simulink model "C1_Full_Car_Model"  (R2023b)
settings: Solver=FixedStepAuto  StartTime=0.0  StopTime=t_end_sim  FixedStep=Ts_sim  RelTol=1e-3
values from neighbouring files (symbols this model uses):
  a_b_ref_sat = [ zeros(1,10) ... (first row only)    [A1_Init.m]    (also in C1_MonteCarloAnalysis.m)
  adaptive = 3    [A1_Init.m]    (also in C1_MonteCarloAnalysis.m = 1)
  data = A2_Full_car_model_parameters_4onBoard()    [A1_Init.m]    (also in C1_MonteCarloAnalysis.m)
  Ft_demand_F = [zeros(1,601) 200*ones(1,2400)]./data.R_F    [A1_Init.m]    (also in C1_MonteCarloAnalysis.m)
  Ft_demand_R = [zeros(1,(601-length(l_discr)))              200*ones(1,(2400+length(l_discr)))]./data.R_R    [A1_Init.m]    (also in C1_MonteCarloAnalysis.m)
  handmade_front = strcat(currentPath,'\Road_profiles\height_crg_files\','handmade_step_3cm_singlefunctions.crg')    [A1_Init.m]    (also in C1_MonteCarloAnalysis.m)
  handmade_mu_front = strcat(currentPath,'\Road_profiles\friction_crg_files\','handmade_fric_step_01_singlefunctions.crg')    [A1_Init.m]    (also in C1_MonteCarloAnalysis.m)
  handmade_mu_rear = handmade_mu_front    [A1_Init.m]    (also in C1_MonteCarloAnalysis.m)
  handmade_rear = handmade_front    [A1_Init.m]    (also in C1_MonteCarloAnalysis.m)
  k_mu = mu_prev_scal_fact(i)    [C1_MonteCarloAnalysis.m]
  k_r = road_height_prev_scal_fact(i)    [C1_MonteCarloAnalysis.m]
  LowLim_Q1 = -10    [A1_Init.m]    (also in C1_MonteCarloAnalysis.m)
  M = N    (= 10)    [A1_Init.m]    (also in C1_MonteCarloAnalysis.m)
  mu_distance = test_distance    [A1_Init.m]    (also in C1_MonteCarloAnalysis.m)
  mu_road = [ones(1,1001), 0.1*ones(1,2000)]    [A1_Init.m]    (also in C1_MonteCarloAnalysis.m)
  N = 10    [A1_Init.m]    (also in C1_MonteCarloAnalysis.m)
  N_iter = 3    [A1_Init.m]    (also in C1_MonteCarloAnalysis.m)
  omega_ini_F_L = x_u_dot_ini_F_L/data.R_F    [A1_Init.m]    (also in C1_MonteCarloAnalysis.m)
  omega_ini_F_R = x_u_dot_ini_R_R/data.R_F    [A1_Init.m]    (also in C1_MonteCarloAnalysis.m)
  omega_ini_R_L = x_u_dot_ini_R_L/data.R_R +2.483*1e-6    [A1_Init.m]    (also in C1_MonteCarloAnalysis.m)
  omega_ini_R_R = x_u_dot_ini_R_R/data.R_R+2.483*1e-6    [A1_Init.m]    (also in C1_MonteCarloAnalysis.m)
  passive = 2    [A1_Init.m]    (also in C1_MonteCarloAnalysis.m)
  Pitch = 0    [A1_Init.m]    (also in C1_MonteCarloAnalysis.m)
  Pitch_dot = 0    [A1_Init.m]    (also in C1_MonteCarloAnalysis.m)
  preview = 2    [A1_Init.m]    (also in C1_MonteCarloAnalysis.m)
  Q1 = 1e6    (= 1000000)    [A1_Init.m]    (also in C1_MonteCarloAnalysis.m)
  Q1_sat = 0    [A1_Init.m]    (also in C1_MonteCarloAnalysis.m)
  Q2 = 1e5    (= 100000)    [A1_Init.m]    (also in C1_MonteCarloAnalysis.m)
  QN1 = 0    [A1_Init.m]    (also in C1_MonteCarloAnalysis.m)
  QN2 = 0    [A1_Init.m]    (also in C1_MonteCarloAnalysis.m)
  R1 = 1e10    (= 10000000000)    [A1_Init.m]    (also in C1_MonteCarloAnalysis.m)
  r1_h0 = 0.99    [A1_Init.m]    (also in C1_MonteCarloAnalysis.m)
  r1_k = 1000    [A1_Init.m]    (also in C1_MonteCarloAnalysis.m)
  r1_max = 11    [A1_Init.m]    (also in C1_MonteCarloAnalysis.m)
  r1_min = -10    [A1_Init.m]    (also in C1_MonteCarloAnalysis.m)
  r2 = 2    [A1_Init.m]    (also in C1_MonteCarloAnalysis.m)
  R2 = 1e2    (= 100)    [A1_Init.m]    (also in C1_MonteCarloAnalysis.m)
  R2_rl = 2    [A1_Init.m]    (also in C1_MonteCarloAnalysis.m)
  road_profile = [zeros(1,801),ones(1,2200)*10*Step_selector]    [A1_Init.m]    (also in C1_MonteCarloAnalysis.m)
  T_distance = test_distance    [A1_Init.m]    (also in C1_MonteCarloAnalysis.m)
  T_hs_ini_F_L = 0    [A1_Init.m]    (also in C1_MonteCarloAnalysis.m)
  T_hs_ini_F_R = 0    [A1_Init.m]    (also in C1_MonteCarloAnalysis.m)
  T_hs_ini_R_L = 0    [A1_Init.m]    (also in C1_MonteCarloAnalysis.m)
  T_hs_ini_R_R = 0    [A1_Init.m]    (also in C1_MonteCarloAnalysis.m)
  test_distance = 0:0.01:30    [A1_Init.m]    (also in C1_MonteCarloAnalysis.m)
  theta_s_ini_F_L = 0    [A1_Init.m]    (also in C1_MonteCarloAnalysis.m)
  theta_s_ini_F_R = 0    [A1_Init.m]    (also in C1_MonteCarloAnalysis.m)
  theta_s_ini_R_L = 0    [A1_Init.m]    (also in C1_MonteCarloAnalysis.m)
  theta_s_ini_R_R = 0    [A1_Init.m]    (also in C1_MonteCarloAnalysis.m)
  theta_w_ini_F_L = -1.056*1e-2    (= -0.01056)    [A1_Init.m]    (also in C1_MonteCarloAnalysis.m)
  theta_w_ini_R_L = -1.056*1e-2    (= -0.01056)    [A1_Init.m]    (also in C1_MonteCarloAnalysis.m)
  Ts = 1e-3*[0 5 10 15 20 25 30 40 60 80 100]    [A1_Init.m]    (also in C1_MonteCarloAnalysis.m)
  w1_h0 = 0.0008    [A1_Init.m]    (also in C1_MonteCarloAnalysis.m)
  w1_k = 5000    [A1_Init.m]    (also in C1_MonteCarloAnalysis.m)
  w1_max = 9    [A1_Init.m]    (also in C1_MonteCarloAnalysis.m)
  w1_min = -10    [A1_Init.m]    (also in C1_MonteCarloAnalysis.m)
  w1_sat = 0.085    [A1_Init.m]    (also in C1_MonteCarloAnalysis.m)
  w2_h0 = 2    [A1_Init.m]    (also in C1_MonteCarloAnalysis.m)
  w2_inc = 0.05    [A1_Init.m]    (also in C1_MonteCarloAnalysis.m)
  w2_k = 10    [A1_Init.m]    (also in C1_MonteCarloAnalysis.m)
  w2_max = 5.3    [A1_Init.m]    (also in C1_MonteCarloAnalysis.m)
  w2_min = -10    [A1_Init.m]    (also in C1_MonteCarloAnalysis.m)
  Wmat_NMPC_init = [W(1,:) W(2,:) W(3,:) W(4,:)]    [A1_Init.m]    (also in C1_MonteCarloAnalysis.m)
  WNmat_NMPC_init = [WN(1,:) WN(2,:)]    [A1_Init.m]    (also in C1_MonteCarloAnalysis.m)
  X_0 = [z_b_dot_ini z_b_ini z_u_dot_ini_F_L z_u_ini_F_L x_b_dot_ini x_b_ini x_u_dot_ini_F_L x_u_ini_F_L          omega_ini_F_L theta_w_ini_F_L omega_ini_F_L theta_s_ini_F_L torque_ini_F_L]    [A1_Init.m]    (also in C1_MonteCarloAnalysis.m)
  x_b_dot_ini = speed_ini/3.6    (= 11.1111111111)    [A1_Init.m]    (also in C1_MonteCarloAnalysis.m)
  x_b_ini = data.b+pos_ini    [A1_Init.m]    (also in C1_MonteCarloAnalysis.m)
  x_err = road_prev_pos_err(i)    [C1_MonteCarloAnalysis.m]
  x_u_dot_ini_F_L = speed_ini/3.6 - 1.125*1e-4    (= 11.1109986111)    [A1_Init.m]    (also in C1_MonteCarloAnalysis.m)
  x_u_dot_ini_F_R = speed_ini/3.6 - 1.125*1e-4    (= 11.1109986111)    [A1_Init.m]    (also in C1_MonteCarloAnalysis.m)
  x_u_dot_ini_R_L = speed_ini/3.6 - 1.125*1e-4    (= 11.1109986111)    [A1_Init.m]    (also in C1_MonteCarloAnalysis.m)
  x_u_dot_ini_R_R = speed_ini/3.6 - 1.125*1e-4    (= 11.1109986111)    [A1_Init.m]    (also in C1_MonteCarloAnalysis.m)
  x_u_ini_F_L = data.a+data.b+pos_ini    [A1_Init.m]    (also in C1_MonteCarloAnalysis.m)
  x_u_ini_F_R = data.a+data.b+pos_ini    [A1_Init.m]    (also in C1_MonteCarloAnalysis.m)
  x_u_ini_R_L = pos_ini    (= 0)    [A1_Init.m]    (also in C1_MonteCarloAnalysis.m)
  x_u_ini_R_R = pos_ini    (= 0)    [A1_Init.m]    (also in C1_MonteCarloAnalysis.m)
  z_b_dot_ini = 0    [A1_Init.m]    (also in C1_MonteCarloAnalysis.m)
  z_b_ini = 0    [A1_Init.m]    (also in C1_MonteCarloAnalysis.m)
  z_u_dot_ini_F_L = 0    [A1_Init.m]    (also in C1_MonteCarloAnalysis.m)
  z_u_dot_ini_F_R = 0    [A1_Init.m]    (also in C1_MonteCarloAnalysis.m)
  z_u_dot_ini_R_L = 0    [A1_Init.m]    (also in C1_MonteCarloAnalysis.m)
  z_u_dot_ini_R_R = 0    [A1_Init.m]    (also in C1_MonteCarloAnalysis.m)
  z_u_ini_F_L = 0    [A1_Init.m]    (also in C1_MonteCarloAnalysis.m)
  z_u_ini_F_R = 0    [A1_Init.m]    (also in C1_MonteCarloAnalysis.m)
  z_u_ini_R_L = 0    [A1_Init.m]    (also in C1_MonteCarloAnalysis.m)
  z_u_ini_R_R = 0    [A1_Init.m]    (also in C1_MonteCarloAnalysis.m)
undefined symbols (not defined in the file or in its folder): Delay_step, road_with_noise
libraries: mfswift_library x8, rllib x4, simulink x4
(part 2 of 7)

== system C1_Full_Car_Model/PASSIVE ==
  BUS : Inport
  Bus Selector : BusSelector  OutputSignals=States.x_u_F_L,States.x_u_F_R,States.x_u_R_L,States.x_u_R_R
  F_t_req1 : Lookup_n-D  NumberOfTableDimensions=1  BreakpointsForDimension1=T_distance  Table=Ft_demand_F  InterpMethod=Linear Lagrange  InternalRulePriority=Speed  RndMeth=Simplest
  F_t_req2 : Lookup_n-D  NumberOfTableDimensions=1  BreakpointsForDimension1=T_distance  Table=Ft_demand_R  InterpMethod=Linear Lagrange  InternalRulePriority=Speed  RndMeth=Simplest
  F_t_req3 : Lookup_n-D  NumberOfTableDimensions=1  BreakpointsForDimension1=T_distance  Table=Ft_demand_R  InterpMethod=Linear Lagrange  InternalRulePriority=Speed  RndMeth=Simplest
  F_t_req4 : Lookup_n-D  NumberOfTableDimensions=1  BreakpointsForDimension1=T_distance  Table=Ft_demand_F  InterpMethod=Linear Lagrange  InternalRulePriority=Speed  RndMeth=Simplest
  Gain : Gain  Gain=data.R_F
  Gain1 : Gain  Gain=data.R_R
  Gain2 : Gain  Gain=data.R_R
  Gain3 : Gain  Gain=data.R_F
  Gain6 : Gain  Gain=1/data.R_F
  Gain7 : Gain  Gain=1/data.R_R
  To Workspace : ToWorkspace  VariableName=T_ref_front_sim  SaveFormat=Timeseries  SampleTime=-1
  To Workspace1 : ToWorkspace  VariableName=T_ref_rear_sim  SaveFormat=Timeseries  SampleTime=-1
  Tt_req_F_L1 : Outport  VectorParamsAs1DForOutWhenUnconnected=off
  Tt_req_F_R1 : Outport  Port=2  VectorParamsAs1DForOutWhenUnconnected=off
  Tt_req_R_L1 : Outport  Port=3  VectorParamsAs1DForOutWhenUnconnected=off
  Tt_req_R_R1 : Outport  Port=4  VectorParamsAs1DForOutWhenUnconnected=off
  tag scope: Ft_req_F=global, Ft_req_R=global
  wires:
  F_t_req1/1 -> Gain/1
  BUS/1 -> Bus Selector/1
  Bus Selector/3 -> F_t_req2/1  "<x_u_R_L>"
  F_t_req2/1 -> Gain1/1
  Bus Selector/1 -> F_t_req1/1  "<x_u_F_L>"
  F_t_req3/1 -> Gain2/1
  Bus Selector/4 -> F_t_req3/1  "<x_u_R_R>"
  Bus Selector/2 -> F_t_req4/1  "<x_u_F_R>"
  F_t_req4/1 -> Gain3/1
  Gain/1 -> Gain6/1, Tt_req_F_L1/1, To Workspace/1
  Gain3/1 -> Tt_req_F_R1/1
  Gain2/1 -> Gain7/1, Tt_req_R_R1/1, To Workspace1/1
  Gain7/1 -> [Ft_req_R]
  Gain1/1 -> Tt_req_R_L1/1
  Gain6/1 -> [Ft_req_F]

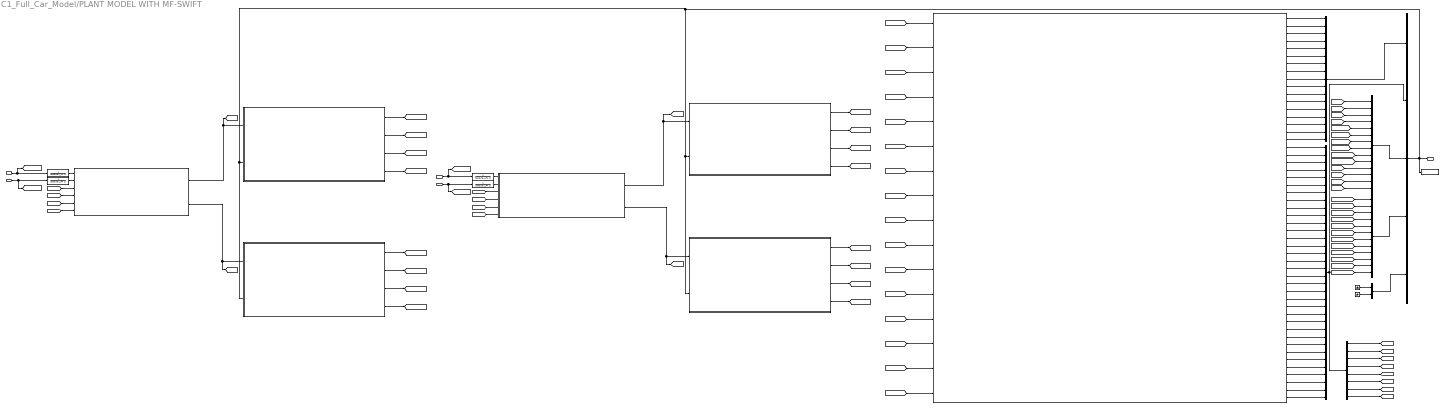
== system C1_Full_Car_Model/PLANT MODEL WITH MF-SWIFT ==
  Tm_F_L_req : Inport
  Tm_F_R_req : Inport  Port=2
  Tm_R_L_req : Inport  Port=3
  Tm_R_R_req : Inport  Port=4
  4 ON-BOARD POWERTRAIN - FRONT : Subsystem
  4 ON-BOARD POWERTRAIN - REAR : Subsystem
  Bus Creator : BusCreator  Inputs=12
  Bus Creator1 : BusCreator  Inputs=17
  Bus Creator2 : BusCreator  Inputs=34
  Bus Creator4 : BusCreator  Inputs=5
  Bus Creator5 : BusCreator  Inputs=14
  Bus Creator6 : BusCreator  Inputs=2
  Bus Selector1 : BusSelector  OutputSignals=omega_R_L,theta_R_L,omega_R_R,theta_R_R,omega_F_L,theta_F_L,omega_F_R,theta_F_R
  FRONT LEFT WHEEL : Subsystem
  FRONT RIGHT WHEEL : Subsystem
  Ground : Ground
  Ground1 : Ground
  MT dynamics1 : TransferFcn  Denominator=[data.tau_R4 1]
  MT dynamics2 : TransferFcn  Denominator=[data.tau_R4 1]
  MT dynamics3 : TransferFcn  Denominator=[data.tau_F4 1]
  MT dynamics4 : TransferFcn  Denominator=[data.tau_F4 1]
  REAR LEFT WHEEL : Subsystem
  REAR RIGHT WHEEL : Subsystem
  SUSPENSION MODEL : Subsystem
  To Workspace : ToWorkspace  VariableName=BUS  SaveFormat=Timeseries  SampleTime=-1
  BUS : Outport  VectorParamsAs1DForOutWhenUnconnected=off
  wires:
  [omega_F_L] -> 4 ON-BOARD POWERTRAIN - FRONT/4(omega_w_L)
  [omega_F_R] -> 4 ON-BOARD POWERTRAIN - FRONT/6(omega_w_R)
  [theta_F_R] -> 4 ON-BOARD POWERTRAIN - FRONT/5(theta_w_R)
  [theta_F_L] -> 4 ON-BOARD POWERTRAIN - FRONT/3(theta_w_L)
  [theta_R_R] -> 4 ON-BOARD POWERTRAIN - REAR/5(theta_w_R)
  [omega_R_R] -> 4 ON-BOARD POWERTRAIN - REAR/6(omega_w_R)
  [omega_R_L] -> 4 ON-BOARD POWERTRAIN - REAR/4(omega_w_L)
  [theta_R_L] -> 4 ON-BOARD POWERTRAIN - REAR/3(theta_w_L)
  [theta_s_ddot_F_R] -> Bus Creator/2  "theta_s_ddot_F_R"
  [theta_s_ddot_F_L] -> Bus Creator/1  "theta_s_ddot_F_L"
  [theta_s_ddot_R_R] -> Bus Creator/8  "theta_s_ddot_R_R"
  [theta_s_R_R] -> Bus Creator/12  "theta_s_R_R"
  [theta_s_R_L] -> Bus Creator/11  "theta_s_R_L"
  [theta_s_ddot_R_L] -> Bus Creator/7  "theta_s_ddot_R_L"
  [theta_s_F_R] -> Bus Creator/6  "theta_s_F_R"
  [theta_s_F_L] -> Bus Creator/5  "theta_s_F_L"
  [theta_s_dot_F_R] -> Bus Creator/4  "theta_s_dot_F_R"
  [theta_s_dot_F_L] -> Bus Creator/3  "theta_s_dot_F_L"
  Bus Creator/1 -> Bus Creator4/4  "Differentials"
  [T_hs_R_L] -> Bus Creator5/11  "T_hs_R_L"
  [T_hs_R_R] -> Bus Creator5/12  "T_hs_R_R"
  [T_hs_F_L] -> Bus Creator5/13  "T_hs_F_L"
  [T_hs_F_R] -> Bus Creator5/14  "T_hs_F_R"
  Bus Selector1/8 -> [theta_F_R]  "<theta_F_R>"
  Bus Selector1/7 -> [omega_F_R]  "<omega_F_R>"
  Bus Selector1/6 -> [theta_F_L]  "<theta_F_L>"
  Bus Selector1/5 -> [omega_F_L]  "<omega_F_L>"
  Bus Selector1/4 -> [theta_R_R]  "<theta_R_R>"
  Bus Selector1/1 -> [omega_R_L]  "<omega_R_L>"
  Bus Selector1/2 -> [theta_R_L]  "<theta_R_L>"
  Bus Selector1/3 -> [omega_R_R]  "<omega_R_R>"
  [Slip_F_R] -> SUSPENSION MODEL/16(Slip_F_R)
  [Rotational_F_R] -> SUSPENSION MODEL/15(Rotational_F_R)
  [Fz_F_R_tot] -> SUSPENSION MODEL/14(Fz_F_R_tot)
  [Fx_F_R] -> SUSPENSION MODEL/13(Fx_F_R)
  [Slip_F_L] -> SUSPENSION MODEL/12(Slip_F_L)
  [Rotational_F_L] -> SUSPENSION MODEL/11(Rotational_F_L)
  [Fz_F_L_tot] -> SUSPENSION MODEL/10(Fz_F_L_tot)
  [Fx_F_L] -> SUSPENSION MODEL/9(Fx_F_L)
  [Slip_R_R] -> SUSPENSION MODEL/8(Slip_R_R)
  [Rotational_R_R] -> SUSPENSION MODEL/7(Rotational_R_R)
  [Fz_R_R_tot] -> SUSPENSION MODEL/6(Fz_R_R_tot)
  [Fx_R_R] -> SUSPENSION MODEL/5(Fx_R_R)
  FRONT LEFT WHEEL/1(Fx_F_L) -> [Fx_F_L]
  FRONT LEFT WHEEL/2(Fz_F_L_tot) -> [Fz_F_L_tot]
  FRONT LEFT WHEEL/3(Rotational_F_L) -> [Rotational_F_L]
  FRONT LEFT WHEEL/4(Slip_F_L) -> [Slip_F_L]
  FRONT RIGHT WHEEL/4(Slip_F_R) -> [Slip_F_R]
  FRONT RIGHT WHEEL/3(Rotational_F_R) -> [Rotational_F_R]
  FRONT RIGHT WHEEL/2(Fz_F_R_tot) -> [Fz_F_R_tot]
  FRONT RIGHT WHEEL/1(Fx_F_R) -> [Fx_F_R]
  REAR RIGHT WHEEL/1(Fx_R_R) -> [Fx_R_R]
  REAR RIGHT WHEEL/2(Fz_R_R_tot) -> [Fz_R_R_tot]
  REAR RIGHT WHEEL/3(Rotational_R_R) -> [Rotational_R_R]
  REAR RIGHT WHEEL/4(Slip_R_R) -> [Slip_R_R]
  REAR LEFT WHEEL/4(Slip_R_L) -> [Slip_R_L]
  REAR LEFT WHEEL/3(Rotational_R_L) -> [Rotational_R_L]
  REAR LEFT WHEEL/2(Fz_R_L_tot) -> [Fz_R_L_tot]
  REAR LEFT WHEEL/1(Fx_R_L) -> [Fx_R_L]
  [Slip_R_L] -> SUSPENSION MODEL/4(Slip_R_L)
  [Rotational_R_L] -> SUSPENSION MODEL/3(Rotational_R_L)
  [Fz_R_L_tot] -> SUSPENSION MODEL/2(Fz_R_L_tot)
  [Fx_R_L] -> SUSPENSION MODEL/1(Fx_R_L)
  SUSPENSION MODEL/38(omega_R_L) -> Bus Creator2/21  "omega_R_L"
  SUSPENSION MODEL/37(x_u_F_R) -> Bus Creator2/20  "x_u_F_R"
  SUSPENSION MODEL/36(x_u_dot_F_R) -> Bus Creator2/19  "x_u_dot_F_R"
  SUSPENSION MODEL/35(x_u_F_L) -> Bus Creator2/18  "x_u_F_L"
  SUSPENSION MODEL/34(x_u_dot_F_L) -> Bus Creator2/17  "x_u_dot_F_L"
  SUSPENSION MODEL/51(slip_F_R) -> Bus Creator2/34  "slip_F_R"
  SUSPENSION MODEL/50(slip_F_L) -> Bus Creator2/33  "slip_F_L"
  SUSPENSION MODEL/49(slip_R_R) -> Bus Creator2/32  "slip_R_R"
  SUSPENSION MODEL/48(slip_R_L) -> Bus Creator2/31  "slip_R_L"
  SUSPENSION MODEL/47(pitch) -> Bus Creator2/30  "pitch"
  SUSPENSION MODEL/46(pitch_dot) -> Bus Creator2/29  "pitch_dot"
  SUSPENSION MODEL/45(theta_F_R) -> Bus Creator2/28  "theta_F_R"
  SUSPENSION MODEL/44(omega_F_R) -> Bus Creator2/27  "omega_F_R"
  SUSPENSION MODEL/43(theta_F_L) -> Bus Creator2/26  "theta_F_L"
  SUSPENSION MODEL/42(omega_F_L) -> Bus Creator2/25  "omega_F_L"
  SUSPENSION MODEL/41(theta_R_R) -> Bus Creator2/24  "theta_R_R"
  SUSPENSION MODEL/40(omega_R_R) -> Bus Creator2/23  "omega_R_R"
  SUSPENSION MODEL/39(theta_R_L) -> Bus Creator2/22  "theta_R_L"
  SUSPENSION MODEL/33(x_u_R_R) -> Bus Creator2/16  "x_u_R_R"
  SUSPENSION MODEL/32(x_u_dot_R_R) -> Bus Creator2/15  "x_u_dot_R_R"
  SUSPENSION MODEL/31(x_u_R_L) -> Bus Creator2/14  "x_u_R_L"
  SUSPENSION MODEL/30(x_u_dot_R_L) -> Bus Creator2/13  "x_u_dot_R_L"
  SUSPENSION MODEL/29(x_b) -> Bus Creator2/12  "x_b"
  SUSPENSION MODEL/28(x_b_dot) -> Bus Creator2/11  "x_b_dot"
  SUSPENSION MODEL/27(z_u_F_R) -> Bus Creator2/10  "z_u_F_R"
  SUSPENSION MODEL/26(z_u_dot_F_R) -> Bus Creator2/9  "z_u_dot_F_R"
  SUSPENSION MODEL/25(z_u_F_L) -> Bus Creator2/8  "z_u_F_L"
  SUSPENSION MODEL/24(z_u_dot_F_L) -> Bus Creator2/7  "z_u_dot_F_L"
  SUSPENSION MODEL/23(z_u_R_R) -> Bus Creator2/6  "z_u_R_R"
  SUSPENSION MODEL/22(z_u_dot_R_R) -> Bus Creator2/5  "z_u_dot_R_R"
  SUSPENSION MODEL/21(z_u_R_L) -> Bus Creator2/4  "z_u_R_L"
  SUSPENSION MODEL/20(z_u_dot_R_L) -> Bus Creator2/3  "z_u_dot_R_L"
  SUSPENSION MODEL/19(z_b) -> Bus Creator2/2  "z_b"
  SUSPENSION MODEL/18(z_b_dot) -> Bus Creator2/1  "z_b_dot"
  SUSPENSION MODEL/17(pitch_ddot) -> Bus Creator1/17  "pitch_ddot"
  SUSPENSION MODEL/16(omega_dot_F_R) -> Bus Creator1/16  "omega_dot_F_R"
  SUSPENSION MODEL/15(omega_dot_F_L) -> Bus Creator1/15  "omega_dot_F_L"
  SUSPENSION MODEL/14(omega_dot_R_R) -> Bus Creator1/14  "omega_dot_R_R"
  SUSPENSION MODEL/13(omega_dot_R_L) -> Bus Creator1/13  "omega_dot_R_L"
  Bus Creator1/1 -> Bus Creator4/1  "Accelerations"
  SUSPENSION MODEL/12(x_u_ddot_F_R) -> Bus Creator1/12  "x_u_ddot_F_R"
  SUSPENSION MODEL/11(x_u_ddot_F_L) -> Bus Creator1/11  "x_u_ddot_F_L"
  SUSPENSION MODEL/10(x_u_ddot_R_R) -> Bus Creator1/10  "x_u_ddot_R_R"
  SUSPENSION MODEL/9(x_u_ddot_R_L) -> Bus Creator1/9  "x_u_ddot_R_L"
  SUSPENSION MODEL/8(jerk) -> Bus Creator1/8  "jerk"
  SUSPENSION MODEL/7(x_b_ddot) -> Bus Creator1/7  "x_b_ddot"
  SUSPENSION MODEL/6(z_u_ddot_F_R) -> Bus Creator1/6  "z_u_ddot_F_R"
  SUSPENSION MODEL/5(z_u_ddot_F_L) -> Bus Creator1/5  "z_u_ddot_F_L"
  SUSPENSION MODEL/4(z_u_ddot_R_R) -> Bus Creator1/4  "z_u_ddot_R_R"
  SUSPENSION MODEL/3(z_u_ddot_R_L) -> Bus Creator1/3  "z_u_ddot_R_L"
  SUSPENSION MODEL/2(jerk_z) -> Bus Creator1/2  "jerk_z"
  SUSPENSION MODEL/1(z_b_ddot) -> Bus Creator1/1  "z_b_ddot"
  [Tm_R_L] -> Bus Creator5/3  "Tm_R_L"
  [Tm_F_R] -> Bus Creator5/2  "Tm_F_R"
  [Ft_req_F] -> Bus Creator5/9  "Ft_F_req"
  [Ft_req_R] -> Bus Creator5/10  "Ft_R_req"
  [Tm_R_R_cor] -> Bus Creator5/8  "Tm_R_R_req"
  Ground1/1 -> Bus Creator6/2  "Fu_R"
  Ground/1 -> Bus Creator6/1  "Fu_F"
  [Tm_F_R_cor] -> Bus Creator5/6  "Tm_F_R_req"
  Bus Creator2/1 -> Bus Creator4/2, Bus Selector1/1  "States"
  Bus Creator6/1 -> Bus Creator4/5  "Act_susp_forces"
  Bus Creator5/1 -> Bus Creator4/3  "Traction_forces"
  [Tm_F_L] -> Bus Creator5/1  "Tm_F_L"
  [Tm_R_R] -> Bus Creator5/4  "Tm_R_R"
  [Tm_F_L_cor] -> Bus Creator5/5  "Tm_F_L_req"
  [Tm_R_L_cor] -> Bus Creator5/7  "Tm_R_L_req"
  [theta_s_dot_R_L] -> Bus Creator/9  "theta_s_dot_R_L"
  [theta_s_dot_R_R] -> Bus Creator/10  "theta_s_dot_R_R"
  Tm_R_R_req/1 -> [Tm_R_R_cor], MT dynamics2/1
  4 ON-BOARD POWERTRAIN - FRONT/1(T_hs_L) -> FRONT LEFT WHEEL/1(Tt_F_L), [T_hs_F_L]  "T_hs_F_L"
  Bus Creator4/1 -> REAR RIGHT WHEEL/2(BUS), REAR LEFT WHEEL/2(BUS), FRONT LEFT WHEEL/2(BUS), FRONT RIGHT WHEEL/2(BUS), BUS/1, To Workspace/1  "From plant"
  4 ON-BOARD POWERTRAIN - REAR/2(T_hs_R) -> [T_hs_R_R], REAR RIGHT WHEEL/1(Tt_R_R)  "T_hs_R_R"
  4 ON-BOARD POWERTRAIN - REAR/1(T_hs_L) -> [T_hs_R_L], REAR LEFT WHEEL/1(Tt_R_L)  "T_hs_R_L"
  Tm_R_L_req/1 -> MT dynamics1/1, [Tm_R_L_cor]
  Tm_F_L_req/1 -> MT dynamics3/1, [Tm_F_L_cor]
  Tm_F_R_req/1 -> MT dynamics4/1, [Tm_F_R_cor]
  4 ON-BOARD POWERTRAIN - FRONT/2(T_hs_R) -> [T_hs_F_R], FRONT RIGHT WHEEL/1(Tt_F_R)
  MT dynamics1/1 -> 4 ON-BOARD POWERTRAIN - REAR/1(T_m_L)
  MT dynamics2/1 -> 4 ON-BOARD POWERTRAIN - REAR/2(T_m_R)
  MT dynamics3/1 -> 4 ON-BOARD POWERTRAIN - FRONT/1(T_m_L)
  MT dynamics4/1 -> 4 ON-BOARD POWERTRAIN - FRONT/2(T_m_R)

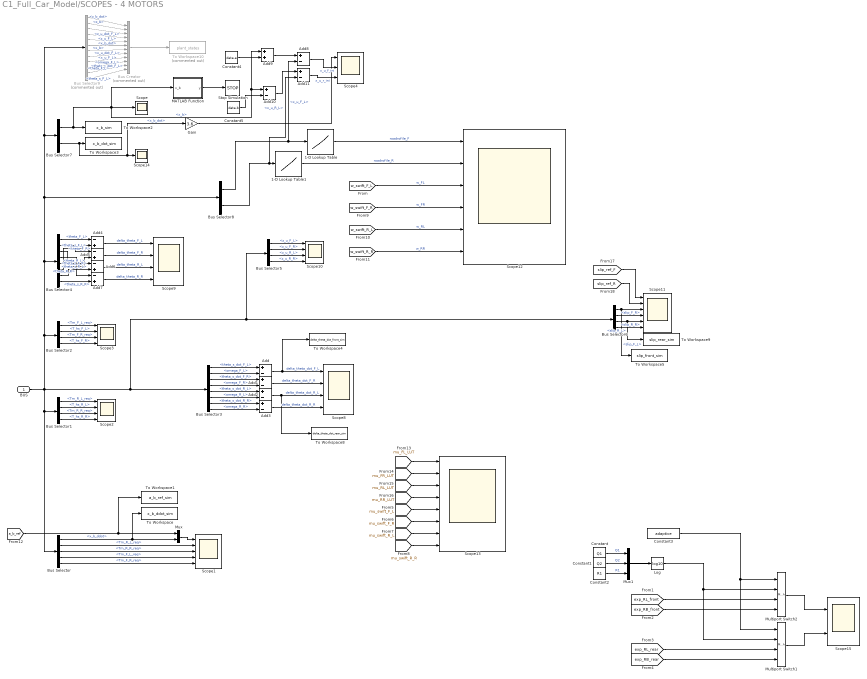
== system C1_Full_Car_Model/SCOPES - 4 MOTORS ==
  BUS : Inport
  1-D Lookup Table : Lookup_n-D  NumberOfTableDimensions=1  BreakpointsForDimension1=test_distance  Table=road_profile*1e-3  InternalRulePriority=Speed  RndMeth=Simplest
  1-D Lookup Table1 : Lookup_n-D  NumberOfTableDimensions=1  BreakpointsForDimension1=test_distance  Table=road_profile*1e-3  InternalRulePriority=Speed  RndMeth=Simplest
  Add{,1..3,8,10..11} (7 alike) : Sum  Inputs=+-
  Add{4..7} (4 alike) : Sum  Inputs=-+
  Add9 : Sum
  Bus Creator : BusCreator  Commented=on  Inputs=12
  Bus Selector : BusSelector  OutputSignals=Accelerations.x_b_ddot,Traction_forces.Tm_R_L_req,Traction_forces.Tm_R_R_req,Traction_forces.Tm_F_L_req,Traction_forces.Tm_F_R_req
  Bus Selector1 : BusSelector  OutputSignals=Traction_forces.Tm_R_L_req,Traction_forces.T_hs_R_L,Traction_forces.Tm_R_R_req,Traction_forces.T_hs_R_R
  Bus Selector2 : BusSelector  OutputSignals=Traction_forces.Tm_F_L_req,Traction_forces.T_hs_F_L,Traction_forces.Tm_F_R_req,Traction_forces.T_hs_F_R
  Bus Selector3 : BusSelector  OutputSignals=Differentials.theta_s_dot_F_L,States.omega_F_L,Differentials.theta_s_dot_F_R,States.omega_F_R,Differentials.theta_s_dot_R_L,States.omega_R_L,Differentials.theta_s_dot_R_R,States.omega_R_R
  Bus Selector4 : BusSelector  OutputSignals=States.theta_F_L,States.theta_F_R,States.theta_R_L,States.theta_R_R,Differentials.theta_s_F_L,Differentials.theta_s_F_R,Differentials.theta_s_R_L,Differentials.theta_s_R_R
  Bus Selector5 : BusSelector  OutputSignals=States.z_u_F_L,States.z_u_F_R,States.z_u_R_L,States.z_u_R_R
  Bus Selector6 : BusSelector  OutputSignals=States.slip_F_L,States.slip_F_R,States.slip_R_L,States.slip_R_R
  Bus Selector7 : BusSelector  OutputSignals=States.x_b,States.x_b_dot
  Bus Selector8 : BusSelector  OutputSignals=States.x_u_F_L,States.x_u_R_L
  Bus Selector9 : BusSelector  Commented=on  OutputSignals=States.z_b_dot,States.z_b,States.z_u_dot_F_L,States.z_u_F_L,States.x_b_dot,States.x_b,States.x_u_dot_F_L,States.x_u_F_L,States.omega_F_L,States.theta_F_L,Differentials.theta_s_dot_F_L,Differentials.theta_s_F_L
  Constant : Constant  Value=Q1
  Constant1 : Constant  Value=Q2
  Constant2 : Constant  Value=R1
  Constant3 : Constant  Value=adaptive
  Constant4 : Constant  Value=data.a
  Constant5 : Constant  Value=data.b
  Gain : Gain  Gain=3.6
  Log : Math  Operator=log10
  MATLAB Function : MATLAB Function  TreatAsAtomicUnit=on
  Multiport Switch1 : MultiPortSwitch  SaturateOnIntegerOverflow=off  InputSameDT=off
  Multiport Switch2 : MultiPortSwitch  SaturateOnIntegerOverflow=off  InputSameDT=off
  Mux : Mux  Inputs=2
  Mux1 : Mux  Inputs=3
  Scope : Scope
  Scope1 : Scope  NumInputPorts=5
  Scope{2..3,8..10} (5 alike) : Scope  NumInputPorts=4
  Scope11 : Scope  NumInputPorts=6
  Scope12 : Scope  NumInputPorts=6
  Scope13 : Scope  NumInputPorts=8
  Scope14 : Scope
  Scope15 : Scope  NumInputPorts=2
  Scope4 : Scope  NumInputPorts=3
  Stop Simulation : Stop
  To Workspace : ToWorkspace  VariableName=x_b_ddot_sim  SaveFormat=Timeseries  SampleTime=-1
  To Workspace1 : ToWorkspace  VariableName=a_b_ref_sim  SaveFormat=Timeseries  SampleTime=-1
  To Workspace10 : ToWorkspace  Commented=on  VariableName=plant_states  SaveFormat=Timeseries  SampleTime=-1
  To Workspace2 : ToWorkspace  VariableName=x_b_sim  SaveFormat=Timeseries  SampleTime=-1
  To Workspace3 : ToWorkspace  VariableName=x_b_dot_sim  SaveFormat=Timeseries  SampleTime=-1
  To Workspace4 : ToWorkspace  VariableName=delta_theta_dot_front_sim  SaveFormat=Timeseries  SampleTime=-1
  To Workspace5 : ToWorkspace  VariableName=slip_front_sim  SaveFormat=Timeseries  SampleTime=-1
  To Workspace8 : ToWorkspace  VariableName=delta_theta_dot_rear_sim  SaveFormat=Timeseries  SampleTime=-1
  To Workspace9 : ToWorkspace  VariableName=slip_rear_sim  SaveFormat=Timeseries  SampleTime=-1
  wires:
  Bus Selector2/4 -> Scope3/4  "<T_hs_F_R>"
  BUS/1 -> Bus Selector5/1, Bus Selector6/1, Bus Selector3/1, Bus Selector1/1, Bus Selector/1, Bus Selector8/1, Bus Selector9/1, Bus Selector7/1, Bus Selector4/1, Bus Selector2/1
  Bus Selector1/4 -> Scope2/4  "<T_hs_R_R>"
  Bus Selector/3 -> Scope1/3  "<Tm_R_R_req>"
  Bus Selector/2 -> Scope1/2  "<Tm_R_L_req>"
  Bus Selector2/1 -> Scope3/1  "<Tm_F_L_req>"
  Bus Selector2/2 -> Scope3/2  "<T_hs_F_L>"
  Bus Selector2/3 -> Scope3/3  "<Tm_F_R_req>"
  Bus Selector1/3 -> Scope2/3  "<Tm_R_R_req>"
  Bus Selector/4 -> Scope1/4  "<Tm_F_L_req>"
  Bus Selector/5 -> Scope1/5  "<Tm_F_R_req>"
  Bus Selector1/2 -> Scope2/2  "<T_hs_R_L>"
  Bus Selector/1 -> To Workspace/1, Mux/2  "<x_b_ddot>"
  Bus Selector1/1 -> Scope2/1  "<Tm_R_L_req>"
  Bus Selector3/1 -> Add/1  "<theta_s_dot_F_L>"
  Bus Selector3/2 -> Add/2  "<omega_F_L>"
  Bus Selector3/3 -> Add1/1  "<theta_s_dot_F_R>"
  Bus Selector3/4 -> Add1/2  "<omega_F_R>"
  Bus Selector3/5 -> Add2/1  "<theta_s_dot_R_L>"
  Bus Selector3/6 -> Add2/2  "<omega_R_L>"
  Bus Selector3/7 -> Add3/1  "<theta_s_dot_R_R>"
  Bus Selector3/8 -> Add3/2  "<omega_R_R>"
  Add/1 -> Scope8/1, To Workspace4/1  "delta_theta_dot_F_L"
  Add1/1 -> Scope8/2  "delta_theta_dot_F_R"
  Add2/1 -> To Workspace8/1, Scope8/3  "delta_theta_dot_R_L"
  Add3/1 -> Scope8/4  "delta_theta_dot_R_R"
  Bus Selector5/1 -> Scope10/1  "<z_u_F_L>"
  Bus Selector5/2 -> Scope10/2  "<z_u_F_R>"
  Bus Selector5/3 -> Scope10/3  "<z_u_R_L>"
  Bus Selector5/4 -> Scope10/4  "<z_u_R_R>"
  Bus Selector6/2 -> Scope11/4  "<slip_F_R>"
  Bus Selector6/3 -> To Workspace9/1, Scope11/5  "<slip_R_L>"
  Bus Selector6/4 -> Scope11/6  "<slip_R_R>"
  Bus Selector6/1 -> To Workspace5/1, Scope11/3  "<slip_F_L>"
  [w_swift_F_R] -> Scope12/4  "w_FR"
  [w_swift_R_L] -> Scope12/5  "w_RL"
  [w_swift_R_R] -> Scope12/6  "w_RR"
  [a_b_ref] -> To Workspace1/1, Mux/1
  Mux/1 -> Scope1/1
  Bus Selector7/1 -> Add10/1, Add9/1, Scope/1, MATLAB Function/1(x_b), To Workspace2/1  "<x_b>"
  Bus Selector7/2 -> Gain/1, Scope14/1, To Workspace3/1  "<x_b_dot>"
  [w_swift_F_L] -> Scope12/3  "w_FL"
  [mu_FL_LUT] -> Scope13/1
  [mu_FR_LUT] -> Scope13/2
  [mu_RL_LUT] -> Scope13/3
  [mu_RR_LUT] -> Scope13/4
  Bus Selector8/1 -> Add8/2, 1-D Lookup Table/1  "<x_u_F_L>"
  Bus Selector8/2 -> Add11/2, 1-D Lookup Table1/1  "<x_u_R_L>"
  1-D Lookup Table/1 -> Scope12/1  "roadrofile_F"
  1-D Lookup Table1/1 -> Scope12/2  "roadrofile_R"
  Bus Creator/1 -> To Workspace10/1
  Bus Selector9/1 -> Bus Creator/1  "<z_b_dot>"
  Bus Selector9/2 -> Bus Creator/2  "<z_b>"
  Bus Selector9/3 -> Bus Creator/3  "<z_u_dot_F_L>"
  Bus Selector9/4 -> Bus Creator/4  "<z_u_F_L>"
  Bus Selector9/5 -> Bus Creator/5  "<x_b_dot>"
  Bus Selector9/6 -> Bus Creator/6  "<x_b>"
  Bus Selector9/7 -> Bus Creator/7  "<x_u_dot_F_L>"
  Bus Selector9/8 -> Bus Creator/8  "<x_u_F_L>"
  Bus Selector9/9 -> Bus Creator/9  "<omega_F_L>"
  Bus Selector9/11 -> Bus Creator/11  "<theta_s_dot_F_L>"
  Bus Selector9/10 -> Bus Creator/10  "<theta_F_L>"
  Bus Selector9/12 -> Bus Creator/12  "<theta_s_F_L>"
  [slip_ref_F] -> Scope11/1
  [slip_ref_R] -> Scope11/2
  MATLAB Function/1(y) -> Stop Simulation/1
  [exp_RL_front] -> Multiport Switch2/3
  Mux1/1 -> Log/1
  Constant/1 -> Mux1/1  "Q1"
  Constant1/1 -> Mux1/2  "Q2"
  Constant2/1 -> Mux1/3  "R1"
  [exp_RB_front] -> Multiport Switch2/4
  Multiport Switch2/1 -> Scope15/1
  Multiport Switch1/1 -> Scope15/2
  [exp_RB_rear] -> Multiport Switch1/4
  [exp_RL_rear] -> Multiport Switch1/3
  Constant3/1 -> Multiport Switch2/1, Multiport Switch1/1
  Bus Selector4/1 -> Add4/1  "<theta_F_L>"
  Bus Selector4/2 -> Add5/1  "<theta_F_R>"
  Bus Selector4/3 -> Add6/1  "<theta_R_L>"
  Bus Selector4/4 -> Add7/1  "<theta_R_R>"
  Bus Selector4/5 -> Add4/2  "<theta_s_F_L>"
  Bus Selector4/6 -> Add5/2  "<theta_s_F_R>"
  Bus Selector4/7 -> Add6/2  "<theta_s_R_L>"
  Bus Selector4/8 -> Add7/2  "<theta_s_R_R>"
  Add4/1 -> Scope9/1  "delta_theta_F_L"
  Add5/1 -> Scope9/2  "delta_theta_F_R"
  Add6/1 -> Scope9/3  "delta_theta_R_L"
  Add7/1 -> Scope9/4  "delta_theta_R_R"
  Add8/1 -> Scope4/2  "x_u_f_ini"
  Constant4/1 -> Add9/2
  Constant5/1 -> Add10/2
  Add11/1 -> Scope4/3  "x_u_r_ini"
  Add9/1 -> Add8/1
  Add10/1 -> Add11/1
  Gain/1 -> Scope4/1
  [mu_swift_F_L] -> Scope13/5
  [mu_swift_F_R] -> Scope13/6
  [mu_swift_R_L] -> Scope13/7
  [mu_swift_R_R] -> Scope13/8
  Log/1 -> Multiport Switch1/2, Multiport Switch2/2

== system C1_Full_Car_Model/CONTROLLER FRONT LEFT/RL_weights ==
  States : Inport
  a_b_ref : Inport  Port=2
  Online Data : Inport  Port=3
  Add : Sum  Inputs=+-
  Add1 : Sum  Inputs=+-
  Add2 : Sum  Inputs=+-
  Bus Selector : BusSelector  OutputSignals=Accelerations.x_b_ddot,Differentials.theta_s_dot_F_L,States.omega_F_L,States.slip_F_L
  Control action : Scope
  Demux : Demux  Commented=on  Outputs=3
  MATLAB Function : MATLAB Function  TreatAsAtomicUnit=on
  MATLAB Function3 : MATLAB Function  TreatAsAtomicUnit=on
  Memory : Memory  InheritSampleTime=on
  Memory1 : Memory  Commented=on  InheritSampleTime=on
  Memory2 : Memory  Commented=on  InheritSampleTime=on
  Memory3 : Memory  Commented=on  InheritSampleTime=on
  Mux : Mux  Commented=on  Inputs=3
  Mux6 : Mux  Inputs=5
  Policy : rllib/Policy  MATFile=blockAgentData_front.mat  SimUsingCodegen=off
  Selector{,1..2,5..6} (5 alike) : Selector  InputPortWidth=1  IndexOptions=Select all  Indices=1  OutputSizes=1
  Subsystem2 : Subsystem
  To Workspace : ToWorkspace  VariableName=exponents_FL_RL  SaveFormat=Timeseries  SampleTime=-1
  Zero-Order Hold : ZeroOrderHold  SampleTime=0.001
  exponents : Outport
  tag scope: exp_RL_front=global
  wires:
  Policy/1 -> Memory/1, Demux/1  "weights"
  Add2/1 -> Selector5/1  "slip_error"
  Bus Selector/4 -> Add2/2  "<slip_F_L>"
  Bus Selector/3 -> Add1/2  "<omega_F_L>"
  Bus Selector/2 -> Add1/1  "<theta_s_dot_F_L>"
  Add1/1 -> Selector6/1  "delta_omega_error"
  Add/1 -> Selector/1  "acc_error"
  Bus Selector/1 -> Add/1  "<x_b_ddot>"
  Subsystem2/3(sigma_ref_act) -> Add2/1
  Subsystem2/2(mu_act_prev) -> MATLAB Function3/1(mu_prev)  "mu_act_prev"
  MATLAB Function3/1(h) -> Selector1/1  "r1"
  MATLAB Function/1(h) -> Selector2/1  "w1"
  Subsystem2/1(w_prev) -> MATLAB Function/1(w_prev)  "w_prev"
  Selector/1 -> Mux6/1
  Selector1/1 -> Mux6/5
  Selector2/1 -> Mux6/4
  Selector5/1 -> Mux6/3
  Selector6/1 -> Mux6/2
  Mux6/1 -> Policy/1
  a_b_ref/1 -> Add/2
  States/1 -> Bus Selector/1
  Online Data/1 -> Subsystem2/1(Online Data)
  Memory1/1 -> Mux/1
  Memory2/1 -> Mux/2
  Memory3/1 -> Mux/3
  Demux/1 -> Memory1/1
  Demux/2 -> Memory2/1
  Demux/3 -> Memory3/1
  Memory/1 -> Control action/1, Zero-Order Hold/1, [exp_RL_front], exponents/1
  Zero-Order Hold/1 -> To Workspace/1

== system C1_Full_Car_Model/CONTROLLER FRONT LEFT/ROAD PREVIEW ==
  F_t : Inport
  CAN : Inport  Port=2
  1-D Lookup Table : Lookup_n-D  NumberOfTableDimensions=1  BreakpointsForDimension1=[0.1:0.1:1]  Table=[0.005 0.01 0.016 0.02 0.025 0.03 0.04 0.05 0.055 0.06]  InternalRulePriority=Speed  RndMeth=Simplest
  1-D Lookup Table1 : Lookup_n-D  NumberOfTableDimensions=1  BreakpointsForDimension1=[0.1:0.1:1]  Table=[0.005 0.01 0.016 0.02 0.025 0.03 0.04 0.05 0.055 0.06]  InternalRulePriority=Speed  RndMeth=Simplest
  1-D Lookup Table2 : Lookup_n-D  NumberOfTableDimensions=1  BreakpointsForDimension1=mu_distance  Table=mu_road  InternalRulePriority=Speed  RndMeth=Simplest
  Bus Selector2 : BusSelector  OutputSignals=States.z_u_F_L
  Bus Selector3 : BusSelector  OutputSignals=States.x_u_F_L,States.x_u_dot_F_L,Traction_forces.Ft_R_req
  Constant : Constant
  Constant1 : Constant  Value=preview
  Constant2 : Constant
  Gain2 : Gain  Gain=data.R_F
  Multiply10 : Gain  Gain=1500/data.Tm_max
  Multiply12 : Gain  Gain=1500/data.Tm_max
  Multiply7 : Gain  Gain=data.R_R
  Multiport Switch2 : MultiPortSwitch  Inputs=2  SaturateOnIntegerOverflow=off  InputSameDT=off
  NO_ROAD_PREVIEW : MATLAB Function  TreatAsAtomicUnit=on
  Product : Product
  Product1 : Product
  ROAD PREVIEW : MATLAB Function  TreatAsAtomicUnit=on
  Time-based Road Preview : Subsystem
  To Workspace : ToWorkspace  VariableName=slip_ref_front_sim  SaveFormat=Timeseries  SampleTime=-1
  To Workspace1 : ToWorkspace  VariableName=mu_front_sim  SaveFormat=Timeseries  SampleTime=-1
  Online Data : Outport
  tag scope: mu_FL_LUT=global, slip_ref_F=global
  wires:
  1-D Lookup Table1/1 -> NO_ROAD_PREVIEW/7(sigma_ref), To Workspace/1, [slip_ref_F]
  1-D Lookup Table/1 -> ROAD PREVIEW/8(sigma_ref)
  ROAD PREVIEW/1(OnlineData) -> Multiport Switch2/3  "Online Data"
  1-D Lookup Table2/1 -> [mu_FL_LUT], To Workspace1/1, NO_ROAD_PREVIEW/6(mu_act), 1-D Lookup Table1/1  "mu_F_L"
  Constant1/1 -> Multiport Switch2/1
  Gain2/1 -> ROAD PREVIEW/3(Tm_req), Multiply12/1, NO_ROAD_PREVIEW/2(Tm_req)
  Bus Selector3/3 -> Product1/1  "<Ft_R_req>"
  F_t/1 -> Gain2/1
  NO_ROAD_PREVIEW/1(OnlineData) -> Multiport Switch2/2  "Online Data"
  Multiply7/1 -> Multiply10/1
  Bus Selector3/1 -> 1-D Lookup Table2/1, Time-based Road Preview/1(x_u)  "<x_u_F_L>"
  Bus Selector3/2 -> Time-based Road Preview/2(x_u_dot)  "<x_u_dot_F_L>"
  Time-based Road Preview/2(beta_y) -> ROAD PREVIEW/2(beta_y)
  Time-based Road Preview/1(w) -> ROAD PREVIEW/1(w)
  Bus Selector2/1 -> NO_ROAD_PREVIEW/1(w)  "<z_u_F_L>"
  Multiport Switch2/1 -> Online Data/1
  CAN/1 -> Bus Selector2/1, Bus Selector3/1
  Product/1 -> NO_ROAD_PREVIEW/3(Tm_req_F2), ROAD PREVIEW/4(Tm_req_F2)
  Time-based Road Preview/3(mu_prev) -> 1-D Lookup Table/1, ROAD PREVIEW/7(mu_act)
  [mu_FL_LUT] -> Product/2
  Product1/1 -> Multiply7/1
  [mu_RL_LUT] -> Product1/2
  Multiply12/1 -> Product/1
  Multiply10/1 -> ROAD PREVIEW/6(Tm_req_R_R), NO_ROAD_PREVIEW/4(Tm_req_R_L), NO_ROAD_PREVIEW/5(Tm_req_R_R), ROAD PREVIEW/5(Tm_req_R_L)

== system C1_Full_Car_Model/CONTROLLER FRONT LEFT/Reference acceleration ==
  Ft : Inport
  x_b_dot : Inport  Port=2
  Ft2 : Inport  Port=3
  2-D Lookup Table : Lookup_n-D  BreakpointsForDimension1=[0:50:350]  BreakpointsForDimension2=[0.1:0.1:1]  Table=a_b_ref_sat  InternalRulePriority=Speed  RndMeth=Simplest
      settings: InputPortMap=u0,u1
  2-D Lookup Table1 : Lookup_n-D  BreakpointsForDimension1=[0:50:350]  BreakpointsForDimension2=[0.1:0.1:1]  Table=a_b_ref_sat  InternalRulePriority=Speed  RndMeth=Simplest
      settings: InputPortMap=u0,u1
  Add : Sum
  Add1 : Sum
  Constant : Constant  Value=-Inf
  Gain : Gain  Gain=0.5
  Gain1 : Gain  Gain=0.5
  Gain2 : Gain  Gain=data.R_F
  Gain3 : Gain  Gain=data.R_R
  Saturation Dynamic : simulink/Discontinuities/Saturation Dynamic  OutMin=[]  OutMax=[]  OutDataTypeStr=Inherit: Same as second input  OutDataType=fixdt(1, 16)  OutScaling=2^-10  DoSatur=off
  a_b_ref : MATLAB Function  TreatAsAtomicUnit=on
  a_ref : Outport
  wires:
  Ft/1 -> Add/1, Gain2/1  "Ft"
  Gain2/1 -> 2-D Lookup Table/1
  Constant/1 -> Saturation Dynamic/3
  Saturation Dynamic/1 -> a_ref/1  "a_b_ref"
  x_b_dot/1 -> a_b_ref/2(vCar_k)  "x_b_dot"
  a_b_ref/1(a_b_ref) -> Saturation Dynamic/2
  Add/1 -> a_b_ref/1(Ft)
  Ft2/1 -> Gain3/1, Add/2  "Ft2"
  Add1/1 -> Saturation Dynamic/1
  Gain3/1 -> 2-D Lookup Table1/1
  [mu_FL_LUT] -> 2-D Lookup Table/2
  [mu_RL_LUT] -> 2-D Lookup Table1/2
  2-D Lookup Table1/1 -> Gain1/1
  2-D Lookup Table/1 -> Gain/1
  Gain/1 -> Add1/1
  Gain1/1 -> Add1/2

== system C1_Full_Car_Model/CONTROLLER FRONT LEFT/Rule based ==
  Online Data : Inport
  BUS : Inport  Port=2
  Flag : Subsystem
  Gain4 : Gain  Gain=data.R_F
  MATLAB Function : MATLAB Function  TreatAsAtomicUnit=on
  MATLAB Function2 : MATLAB Function  TreatAsAtomicUnit=on
  MATLAB Function3 : MATLAB Function  TreatAsAtomicUnit=on
  Min : MinMax  Inputs=2
  Mux : Mux  Inputs=3
  Product : Product
  Selector : Selector  NumberOfDimensions=2  InputPortWidth=1  IndexOptions=Index vector (dialog),Select all  Indices=1,1  OutputSizes=1,1
  Subsystem : Subsystem
  To Workspace9 : ToWorkspace  VariableName=exponents_FL_RB  SaveFormat=Timeseries  SampleTime=-1
  Zero-Order Hold : ZeroOrderHold  SampleTime=0.001
  memory : Subsystem
  exponents : Outport
  tag scope: exp_RB_front=global
  wires:
  Min/1 -> MATLAB Function/2(mu)
  [mu_RL_LUT] -> Min/1
  MATLAB Function3/1(W) -> Mux/3  "r1"
  Subsystem/1(w_prev) -> MATLAB Function/1(w_prev)  "w_prev"
  Selector/1 -> Min/2, Product/1, MATLAB Function2/2(mu)
  Gain4/1 -> memory/1(In1)
  memory/1(Out1) -> MATLAB Function2/1(dT_req)
  Subsystem/2(mu_act_prev) -> Selector/1, Flag/2(mu_prev), MATLAB Function3/2(mu_prev)  "mu_act_prev"
  [Ft_req_F] -> Product/2
  Online Data/1 -> Subsystem/1(Online Data)
  MATLAB Function2/1(W) -> Mux/2  "w2"
  MATLAB Function/1(W) -> Mux/1  "w1"
  Mux/1 -> exponents/1, [exp_RB_front], Zero-Order Hold/1
  Zero-Order Hold/1 -> To Workspace9/1
  Product/1 -> Gain4/1
  BUS/1 -> Flag/1(Measurement data)
  Flag/1(Flag) -> MATLAB Function3/1(flag)

== system C1_Full_Car_Model/CONTROLLER FRONT LEFT/Subsystem1 ==
  exponents : Inport
  Constant : Constant  Value=R2_rl
  Constant1 : Constant  Value=0
  Demux : Demux  Outputs=3
  Exp{,1..3} (4 alike) : Math  Operator=10^u
  MATLAB Function : MATLAB Function  TreatAsAtomicUnit=on
  MATLAB Function1 : MATLAB Function  TreatAsAtomicUnit=on
  MATLAB Function2 : MATLAB Function  TreatAsAtomicUnit=on
  Min : MinMax  Inputs=2
  stage cost matrix : Outport
  terminal cost matrix : Outport  Port=2
  wires:
  MATLAB Function/1(Wmat_NMPC) -> stage cost matrix/1
  MATLAB Function1/1(WNmat_NMPC) -> terminal cost matrix/1
  exponents/1 -> Demux/1
  Demux/1 -> MATLAB Function2/1(Q1)
  Demux/2 -> Exp1/1
  Demux/3 -> Exp2/1
  Exp/1 -> MATLAB Function/1(Q1)
  Exp1/1 -> MATLAB Function/2(Q2)
  Exp2/1 -> MATLAB Function/3(R1)
  Constant/1 -> Exp3/1
  Exp3/1 -> MATLAB Function/4(R2)
  Constant1/1 -> MATLAB Function1/2(QN2), MATLAB Function1/1(QN1)
  [mu_FL_LUT] -> Min/1
  [mu_RL_LUT] -> Min/2
  Min/1 -> MATLAB Function2/2(mu)
  MATLAB Function2/1(Q1_out) -> Exp/1

== system C1_Full_Car_Model/CONTROLLER FRONT LEFT/Subsystem2 ==
  exponents : Inport
  Constant : Constant  Value=r2
  Constant1 : Constant  Value=0
  Demux : Demux  Outputs=3
  Exp{,1..4} (5 alike) : Math  Operator=10^u
  MATLAB Function : MATLAB Function  TreatAsAtomicUnit=on
  MATLAB Function1 : MATLAB Function  TreatAsAtomicUnit=on
  stage cost matrix : Outport
  terminal cost matrix : Outport  Port=2
  wires:
  MATLAB Function1/1(WNmat_NMPC) -> terminal cost matrix/1
  exponents/1 -> Demux/1
  Demux/1 -> Exp/1
  Demux/2 -> Exp1/1
  Demux/3 -> Exp2/1
  Exp/1 -> MATLAB Function/1(Q1)
  Exp1/1 -> MATLAB Function/2(Q2)
  Exp2/1 -> MATLAB Function/3(R1)
  Constant/1 -> Exp3/1
  Exp3/1 -> MATLAB Function/4(R2)
  Constant1/1 -> Exp4/1
  Exp4/1 -> MATLAB Function1/2(QN2), MATLAB Function1/1(QN1)
  MATLAB Function/1(Wmat_NMPC) -> stage cost matrix/1

== system C1_Full_Car_Model/CONTROLLER FRONT LEFT/Weight matrixes ==
  x_u : Inport
  MATLAB Function : MATLAB Function  TreatAsAtomicUnit=on
  Q1 : Lookup_n-D  NumberOfTableDimensions=1  BreakpointsForDimension1=[0 1e6]  Table=[Q1 Q1]  InternalRulePriority=Speed  RndMeth=Simplest
  Q2 : Lookup_n-D  NumberOfTableDimensions=1  BreakpointsForDimension1=[0 1e6]  Table=[Q2 Q2]  InternalRulePriority=Speed  RndMeth=Simplest
  QN1 : Lookup_n-D  NumberOfTableDimensions=1  BreakpointsForDimension1=[0 1e6]  Table=[QN1 QN1]  InternalRulePriority=Speed  RndMeth=Simplest
  QN2 : Lookup_n-D  NumberOfTableDimensions=1  BreakpointsForDimension1=[0 1e6]  Table=[QN2 QN2]  InternalRulePriority=Speed  RndMeth=Simplest
  R1 : Lookup_n-D  NumberOfTableDimensions=1  BreakpointsForDimension1=[0 1e6]  Table=[R1 R1]  InternalRulePriority=Speed  RndMeth=Simplest
  R2 : Lookup_n-D  NumberOfTableDimensions=1  BreakpointsForDimension1=[0 1e6]  Table=[R2 R2]  InternalRulePriority=Speed  RndMeth=Simplest
  Scope : Scope
  Stage Cost Matrix : Outport
  Terminal Cost Matrix : Outport  Port=2
  wires:
  QN2/1 -> MATLAB Function/4(QN2)  "QN2"
  QN1/1 -> MATLAB Function/3(QN1)  "QN1"
  R2/1 -> MATLAB Function/6(R2)  "R2"
  R1/1 -> MATLAB Function/5(R1)  "R1"
  Q2/1 -> MATLAB Function/2(Q2)  "Q2"
  Q1/1 -> MATLAB Function/1(Q1)  "Q1"
  x_u/1 -> R2/1, R1/1, QN2/1, QN1/1, Q2/1, Q1/1
  MATLAB Function/2(WNmat_NMPC) -> Terminal Cost Matrix/1
  MATLAB Function/1(Wmat_NMPC) -> Stage Cost Matrix/1, Scope/1

== system C1_Full_Car_Model/CONTROLLER FRONT RIGHT/RL_weights ==
  States : Inport
  Online Data : Inport  Port=2
  a_b_ref : Inport  Port=3
  Add : Sum  Inputs=+-
  Add1 : Sum  Inputs=+-
  Add2 : Sum  Inputs=+-
  Bus Selector : BusSelector  OutputSignals=Accelerations.x_b_ddot,Differentials.theta_s_dot_F_R,States.omega_F_R,States.slip_F_R
  Control action : Scope
  Demux : Demux  Commented=on  Outputs=3
  MATLAB Function : MATLAB Function  TreatAsAtomicUnit=on
  MATLAB Function3 : MATLAB Function  TreatAsAtomicUnit=on
  Memory1 : Memory  Commented=on  InheritSampleTime=on
  Memory2 : Memory  InheritSampleTime=on
  Memory4 : Memory  Commented=on  InheritSampleTime=on
  Memory5 : Memory  Commented=on  InheritSampleTime=on
  Mux : Mux  Commented=on  Inputs=3
  Mux6 : Mux  Inputs=5
  Policy : rllib/Policy  MATFile=blockAgentData_front.mat  SimUsingCodegen=off
  Selector{,1..2,4..5} (5 alike) : Selector  InputPortWidth=1  IndexOptions=Select all  Indices=1  OutputSizes=1
  Subsystem2 : Subsystem
  exponents : Outport
  wires:
  Mux6/1 -> Policy/1
  Bus Selector/1 -> Add/1  "<x_b_ddot>"
  Add/1 -> Selector/1  "acc_error"
  Add1/1 -> Selector1/1  "delta_omega_error"
  Bus Selector/2 -> Add1/1  "<theta_s_dot_F_R>"
  Bus Selector/3 -> Add1/2  "<omega_F_R>"
  Bus Selector/4 -> Add2/2  "<slip_F_R>"
  Add2/1 -> Selector2/1  "slip_error"
  MATLAB Function3/1(h) -> Selector5/1  "r1"
  MATLAB Function/1(h) -> Selector4/1  "w1"
  Memory2/1 -> exponents/1, Control action/1
  Selector/1 -> Mux6/1  "w1"
  Selector1/1 -> Mux6/2  "w1"
  Selector2/1 -> Mux6/3  "w1"
  Selector4/1 -> Mux6/4  "w1"
  Selector5/1 -> Mux6/5  "w1"
  States/1 -> Bus Selector/1
  Online Data/1 -> Subsystem2/1(Online Data)
  a_b_ref/1 -> Add/2
  Demux/1 -> Memory1/1
  Policy/1 -> Memory2/1, Demux/1  "weights"
  Demux/3 -> Memory5/1
  Memory4/1 -> Mux/2
  Demux/2 -> Memory4/1
  Mux/1 -> ?
  Memory5/1 -> Mux/3
  Memory1/1 -> Mux/1
  Subsystem2/1(w_prev) -> MATLAB Function/1(w_prev)  "w_prev"
  Subsystem2/3(sigma_ref_act) -> Add2/1
  Subsystem2/2(mu_act_prev) -> MATLAB Function3/1(mu_prev)  "mu_act_prev"

== system C1_Full_Car_Model/CONTROLLER FRONT RIGHT/ROAD PREVIEW ==
  F_t : Inport
  CAN : Inport  Port=2
  1-D Lookup Table : Lookup_n-D  NumberOfTableDimensions=1  BreakpointsForDimension1=[0.1:0.1:1]  Table=[0.005 0.01 0.016 0.02 0.025 0.03 0.04 0.05 0.055 0.06]  InternalRulePriority=Speed  RndMeth=Simplest
  1-D Lookup Table1 : Lookup_n-D  NumberOfTableDimensions=1  BreakpointsForDimension1=[0.1:0.1:1]  Table=[0.005 0.01 0.016 0.02 0.025 0.03 0.04 0.05 0.055 0.06]  InternalRulePriority=Speed  RndMeth=Simplest
  1-D Lookup Table2 : Lookup_n-D  NumberOfTableDimensions=1  BreakpointsForDimension1=mu_distance  Table=mu_road  InternalRulePriority=Speed  RndMeth=Simplest
  Bus Selector2 : BusSelector  OutputSignals=States.z_u_F_R
  Bus Selector3 : BusSelector  OutputSignals=States.x_u_F_R,States.x_u_dot_F_R,Traction_forces.Ft_R_req
  Constant : Constant
  Constant1 : Constant  Value=preview
  Constant2 : Constant
  Gain1 : Gain  Gain=data.R_F
  Multiply1 : Gain  Gain=data.R_R
  Multiply10 : Gain  Gain=1500/data.Tm_max
  Multiply12 : Gain  Gain=1500/data.Tm_max
  Multiport Switch2 : MultiPortSwitch  Inputs=2  SaturateOnIntegerOverflow=off  InputSameDT=off
  NO_ROAD_PREVIEW : MATLAB Function  TreatAsAtomicUnit=on
  Product : Product
  Product1 : Product
  ROAD PREVIEW : MATLAB Function  TreatAsAtomicUnit=on
  Time-based Road Preview : Subsystem
  Online Data : Outport
  tag scope: mu_FR_LUT=global
  wires:
  1-D Lookup Table1/1 -> NO_ROAD_PREVIEW/7(sigma_ref)
  Time-based Road Preview/3(mu_prev) -> 1-D Lookup Table/1, ROAD PREVIEW/7(mu_act)  "mu_act"
  Product/1 -> NO_ROAD_PREVIEW/3(Tm_req_F2), NO_ROAD_PREVIEW/5(Tm_req_R_R), ROAD PREVIEW/4(Tm_req_F2)
  CAN/1 -> Bus Selector2/1, Bus Selector3/1
  Multiport Switch2/1 -> Online Data/1
  Bus Selector2/1 -> NO_ROAD_PREVIEW/1(w)  "<z_u_F_R>"
  Time-based Road Preview/1(w) -> ROAD PREVIEW/1(w)
  Time-based Road Preview/2(beta_y) -> ROAD PREVIEW/2(beta_y)
  1-D Lookup Table/1 -> ROAD PREVIEW/8(sigma_ref)
  ROAD PREVIEW/1(OnlineData) -> Multiport Switch2/3  "Online Data"
  Bus Selector3/2 -> Time-based Road Preview/2(x_u_dot)  "<x_u_dot_F_R>"
  Multiply1/1 -> Multiply10/1
  NO_ROAD_PREVIEW/1(OnlineData) -> Multiport Switch2/2  "Online Data"
  Bus Selector3/3 -> Product1/1  "<Ft_R_req>"
  Gain1/1 -> ROAD PREVIEW/3(Tm_req), Multiply12/1, NO_ROAD_PREVIEW/2(Tm_req)
  Multiply10/1 -> ROAD PREVIEW/6(Tm_req_R_R), NO_ROAD_PREVIEW/4(Tm_req_R_L), ROAD PREVIEW/5(Tm_req_R_L)
  Constant1/1 -> Multiport Switch2/1
  1-D Lookup Table2/1 -> [mu_FR_LUT], 1-D Lookup Table1/1, NO_ROAD_PREVIEW/6(mu_act)  "mu_F_R"
  [mu_RL_LUT] -> Product1/2
  [mu_FL_LUT] -> Product/2
  Product1/1 -> Multiply1/1
  F_t/1 -> Gain1/1
  Multiply12/1 -> Product/1
  Bus Selector3/1 -> 1-D Lookup Table2/1, Time-based Road Preview/1(x_u)  "<x_u_F_R>"

== system C1_Full_Car_Model/CONTROLLER FRONT RIGHT/Reference acceleration ==
  Ft : Inport
  x_b_dot : Inport  Port=2
  Ft2 : Inport  Port=3
  2-D Lookup Table : Lookup_n-D  BreakpointsForDimension1=[0:50:350]  BreakpointsForDimension2=[0.1:0.1:1]  Table=a_b_ref_sat  InternalRulePriority=Speed  RndMeth=Simplest
      settings: InputPortMap=u0,u1
  2-D Lookup Table1 : Lookup_n-D  BreakpointsForDimension1=[0:50:350]  BreakpointsForDimension2=[0.1:0.1:1]  Table=a_b_ref_sat  InternalRulePriority=Speed  RndMeth=Simplest
      settings: InputPortMap=u0,u1
  Add : Sum
  Add1 : Sum
  Constant : Constant  Value=-Inf
  Gain : Gain  Gain=0.5
  Gain1 : Gain  Gain=0.5
  Gain2 : Gain  Gain=data.R_F
  Gain3 : Gain  Gain=data.R_R
  Saturation Dynamic : simulink/Discontinuities/Saturation Dynamic  OutMin=[]  OutMax=[]  OutDataTypeStr=Inherit: Same as second input  OutDataType=fixdt(1, 16)  OutScaling=2^-10  DoSatur=off
  a_b_ref : MATLAB Function  TreatAsAtomicUnit=on
  a_ref : Outport
  wires:
  Ft/1 -> Add/1, Gain2/1  "Ft"
  Gain2/1 -> 2-D Lookup Table/1
  Constant/1 -> Saturation Dynamic/3
  Saturation Dynamic/1 -> a_ref/1  "a_b_ref"
  x_b_dot/1 -> a_b_ref/2(vCar_k)  "x_b_dot"
  a_b_ref/1(a_b_ref) -> Saturation Dynamic/2
  Add/1 -> a_b_ref/1(Ft)
  Ft2/1 -> Gain3/1, Add/2  "Ft2"
  Add1/1 -> Saturation Dynamic/1
  Gain3/1 -> 2-D Lookup Table1/1
  [mu_FL_LUT] -> 2-D Lookup Table/2
  [mu_RL_LUT] -> 2-D Lookup Table1/2
  2-D Lookup Table1/1 -> Gain1/1
  2-D Lookup Table/1 -> Gain/1
  Gain/1 -> Add1/1
  Gain1/1 -> Add1/2

== system C1_Full_Car_Model/CONTROLLER FRONT RIGHT/Rule based ==
  Online Data : Inport
  BUS : Inport  Port=2
  Flag : Subsystem
  Gain4 : Gain  Gain=data.R_F
  MATLAB Function : MATLAB Function  TreatAsAtomicUnit=on
  MATLAB Function2 : MATLAB Function  TreatAsAtomicUnit=on
  MATLAB Function3 : MATLAB Function  TreatAsAtomicUnit=on
  Min : MinMax  Inputs=2
  Mux : Mux  Inputs=3
  Product : Product
  Selector : Selector  NumberOfDimensions=2  InputPortWidth=1  IndexOptions=Index vector (dialog),Select all  Indices=1,1  OutputSizes=1,1
  Subsystem : Subsystem
  memory : Subsystem
  exponents : Outport
  wires:
  Min/1 -> MATLAB Function/2(mu)
  [mu_RL_LUT] -> Min/1
  MATLAB Function3/1(W) -> Mux/3  "r1"
  Subsystem/1(w_prev) -> MATLAB Function/1(w_prev)  "w_prev"
  Selector/1 -> Min/2, Product/1, MATLAB Function2/2(mu)
  Gain4/1 -> memory/1(In1)
  memory/1(Out1) -> MATLAB Function2/1(dT_req)
  [Ft_req_F] -> Product/2
  Online Data/1 -> Subsystem/1(Online Data)
  MATLAB Function2/1(W) -> Mux/2  "w2"
  MATLAB Function/1(W) -> Mux/1  "w1"
  Mux/1 -> exponents/1
  Product/1 -> Gain4/1
  Flag/1(Flag) -> MATLAB Function3/1(flag)
  Subsystem/2(mu_act_prev) -> Flag/2(mu_prev), MATLAB Function3/2(mu_prev), Selector/1  "mu_act_prev"
  BUS/1 -> Flag/1(Measurement data)

== system C1_Full_Car_Model/CONTROLLER FRONT RIGHT/Subsystem1 ==
  exponents : Inport
  Constant : Constant  Value=R2_rl
  Constant1 : Constant  Value=0
  Demux : Demux  Outputs=3
  Exp{,1..3} (4 alike) : Math  Operator=10^u
  MATLAB Function : MATLAB Function  TreatAsAtomicUnit=on
  MATLAB Function1 : MATLAB Function  TreatAsAtomicUnit=on
  MATLAB Function2 : MATLAB Function  TreatAsAtomicUnit=on
  Min : MinMax  Inputs=2
  stage cost matrix : Outport
  terminal cost matrix : Outport  Port=2
  wires:
  MATLAB Function/1(Wmat_NMPC) -> stage cost matrix/1
  MATLAB Function1/1(WNmat_NMPC) -> terminal cost matrix/1
  exponents/1 -> Demux/1
  Demux/1 -> MATLAB Function2/1(Q1)
  Demux/2 -> Exp1/1
  Demux/3 -> Exp2/1
  Exp/1 -> MATLAB Function/1(Q1)
  Exp1/1 -> MATLAB Function/2(Q2)
  Exp2/1 -> MATLAB Function/3(R1)
  Constant/1 -> Exp3/1
  Exp3/1 -> MATLAB Function/4(R2)
  Constant1/1 -> MATLAB Function1/2(QN2), MATLAB Function1/1(QN1)
  [mu_FL_LUT] -> Min/1
  [mu_RL_LUT] -> Min/2
  Min/1 -> MATLAB Function2/2(mu)
  MATLAB Function2/1(Q1_out) -> Exp/1

== system C1_Full_Car_Model/CONTROLLER FRONT RIGHT/Subsystem2 ==
  exponents : Inport
  Constant : Constant  Value=r2
  Constant1 : Constant  Value=0
  Demux : Demux  Outputs=3
  Exp{,1..4} (5 alike) : Math  Operator=10^u
  MATLAB Function : MATLAB Function  TreatAsAtomicUnit=on
  MATLAB Function1 : MATLAB Function  TreatAsAtomicUnit=on
  stage cost matrix : Outport
  terminal cost matrix : Outport  Port=2
  wires:
  MATLAB Function/1(Wmat_NMPC) -> stage cost matrix/1
  MATLAB Function1/1(WNmat_NMPC) -> terminal cost matrix/1
  exponents/1 -> Demux/1
  Demux/1 -> Exp/1
  Demux/2 -> Exp1/1
  Demux/3 -> Exp2/1
  Exp/1 -> MATLAB Function/1(Q1)
  Exp1/1 -> MATLAB Function/2(Q2)
  Exp2/1 -> MATLAB Function/3(R1)
  Constant/1 -> Exp3/1
  Exp3/1 -> MATLAB Function/4(R2)
  Constant1/1 -> Exp4/1
  Exp4/1 -> MATLAB Function1/2(QN2), MATLAB Function1/1(QN1)
